simulink model "akgoz_gimbal_stabilized"  (R2025b)
settings: Solver=ode15s  StartTime=0.0  StopTime=12  MaxStep=5e-4  RelTol=1e-5
values from neighbouring files (symbols this model uses):
  kg = gain([a '_kt'],kt(k),[1500 y+120 1550 y+150]); w(is,1,kg,1)    [akgoz_build_controller.m]
  m = akgoz_plot_los(out,['AKGOZ LOS: ' cfg{k,1}])    [akgoz_compare.m]    (also in akgoz_gyro.m = round(m/P.gyro.quant)*P.gyro.quant)
  s = diagSig{r,k}; w(s{1},s{2},dm,n)    [akgoz_build_controller.m]    (also in akgoz_los_kinematics.m = norm(c))
undefined symbols (not defined in the file or in its folder): DiscIntNeverNeededParam, X, Y, Z
libraries: sm_lib x154, nesl_utility x13, simulink x2
(part 1 of 3)
settings Model: Creator=yagiz  LastModifiedBy=yagiz

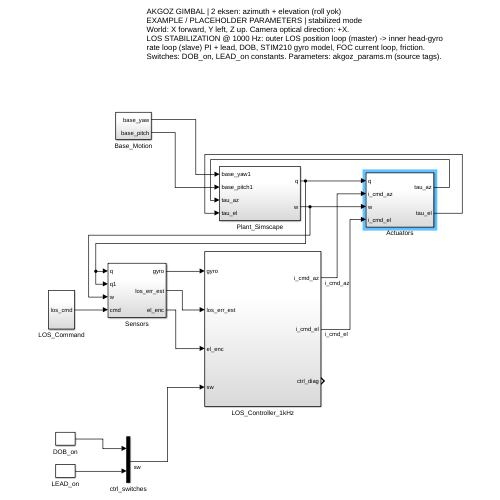
[thumbnail: Simulink's stored preview of the top-level diagram]
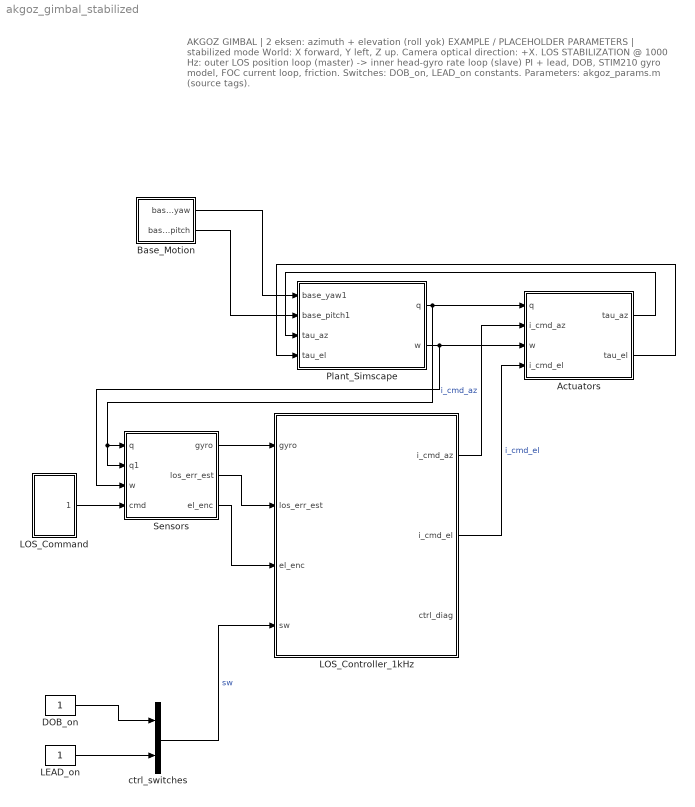
== system akgoz_gimbal_stabilized ==
  note: AKGOZ GIMBAL | 2 eksen: azimuth + elevation (roll yok)
      | EXAMPLE / PLACEHOLDER PARAMETERS | stabilized mode
      | World: X forward, Y left, Z up. Camera optical direction: +X.
      | LOS STABILIZATION @ 1000 Hz: outer LOS position loop (master) -> inner head-gyro
      | rate loop (slave) PI + lead, DOB, STIM210 gyro model, FOC current loop, friction.
      | Switches: DOB_on, LEAD_on constants. Parameters: akgoz_params.m (source tags).
  Actuators : Subsystem
  Base_Motion : Subsystem
  DOB_on : Constant
  LEAD_on : Constant
  LOS_Command : Subsystem
  LOS_Controller_1kHz : Subsystem
  Plant_Simscape : Subsystem
  Sensors : Subsystem
  ctrl_switches : Mux  Inputs=2
  wires:
  DOB_on/1 -> ctrl_switches/1
  LEAD_on/1 -> ctrl_switches/2
  Base_Motion/1(base_yaw) -> Plant_Simscape/1(base_yaw1)
  Actuators/2(tau_el) -> Plant_Simscape/4(tau_el)
  LOS_Command/1(los_cmd) -> Sensors/4(cmd)
  Base_Motion/2(base_pitch) -> Plant_Simscape/2(base_pitch1)
  Sensors/1(gyro) -> LOS_Controller_1kHz/1(gyro)
  Sensors/3(el_enc) -> LOS_Controller_1kHz/3(el_enc)
  Sensors/2(los_err_est) -> LOS_Controller_1kHz/2(los_err_est)
  Plant_Simscape/1(q) -> Sensors/1(q), Sensors/2(q1), Actuators/1(q)
  Plant_Simscape/2(w) -> Actuators/3(w), Sensors/3(w)
  ctrl_switches/1 -> LOS_Controller_1kHz/4(sw)  "sw"
  LOS_Controller_1kHz/1(i_cmd_az) -> Actuators/2(i_cmd_az)  "i_cmd_az"
  Actuators/1(tau_az) -> Plant_Simscape/3(tau_az)
  LOS_Controller_1kHz/2(i_cmd_el) -> Actuators/4(i_cmd_el)  "i_cmd_el"

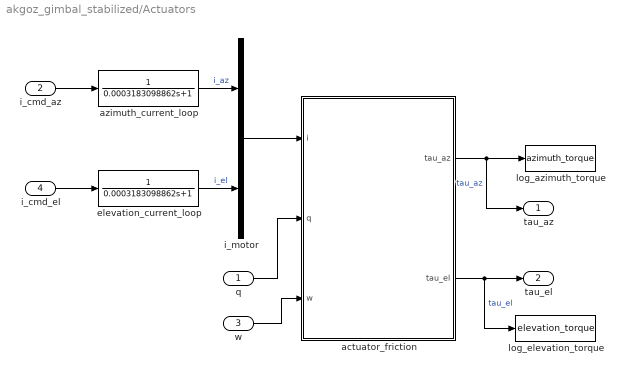
== system akgoz_gimbal_stabilized/Actuators ==
  q : Inport
  i_cmd_az : Inport  Port=2
  w : Inport  Port=3
  i_cmd_el : Inport  Port=4
  actuator_friction : MATLAB Function  TreatAsAtomicUnit=on
  azimuth_current_loop : TransferFcn  Numerator=1  Denominator=[0.0003183098862 1]
  elevation_current_loop : TransferFcn  Numerator=1  Denominator=[0.0003183098862 1]
  i_motor : Mux  Inputs=2
  log_azimuth_torque : ToWorkspace  VariableName=azimuth_torque  SaveFormat=Timeseries  SampleTime=-1
  log_elevation_torque : ToWorkspace  VariableName=elevation_torque  SaveFormat=Timeseries  SampleTime=-1
  tau_az : Outport
  tau_el : Outport  Port=2
  wires:
  actuator_friction/2(tau_el) -> tau_el/1, log_elevation_torque/1  "tau_el"
  actuator_friction/1(tau_az) -> tau_az/1, log_azimuth_torque/1  "tau_az"
  q/1 -> actuator_friction/2(q)
  w/1 -> actuator_friction/3(w)
  i_motor/1 -> actuator_friction/1(i)
  elevation_current_loop/1 -> i_motor/2  "i_el"
  azimuth_current_loop/1 -> i_motor/1  "i_az"
  i_cmd_el/1 -> elevation_current_loop/1
  i_cmd_az/1 -> azimuth_current_loop/1

== system akgoz_gimbal_stabilized/Base_Motion ==
  base_demux : Demux  Outputs=2
  base_motion : MATLAB Function  TreatAsAtomicUnit=on
  clock : Clock
  base_yaw : Outport
  base_pitch : Outport  Port=2
  wires:
  base_demux/2 -> base_pitch/1  "base_pitch"
  base_demux/1 -> base_yaw/1  "base_yaw"
  base_motion/1(y) -> base_demux/1
  clock/1 -> base_motion/1(t)

== system akgoz_gimbal_stabilized/LOS_Command ==
  LOS_az_cmd : Step  Time=6  After=0.2617993877991494  SampleTime=0.001
  LOS_cmd : Mux  Inputs=2
  LOS_el_cmd : Step  Time=2  After=-0.3490658503988659  SampleTime=0.001
  los_cmd : Outport
  wires:
  LOS_cmd/1 -> los_cmd/1  "los_cmd"
  LOS_el_cmd/1 -> LOS_cmd/2
  LOS_az_cmd/1 -> LOS_cmd/1

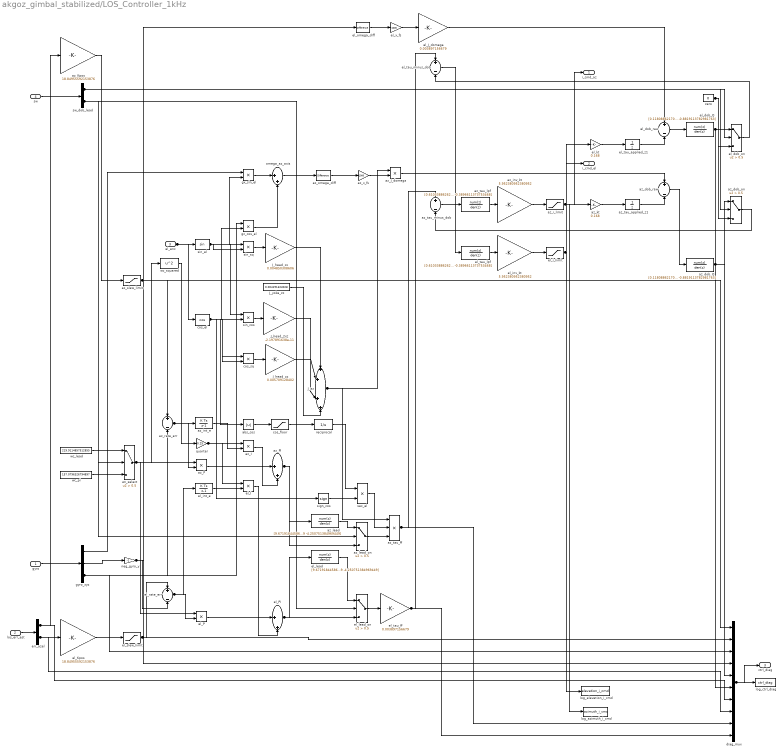
== system akgoz_gimbal_stabilized/LOS_Controller_1kHz ==
  gyro : Inport
  los_err_est : Inport  Port=2
  el_enc : Inport  Port=3
  sw : Inport  Port=4
  J_az : Sum  Inputs=++++
  J_head_2xz : Gain  Gain=-2.197891638e-11
  J_head_xx : Gain  Gain=0.004850308606
  J_head_zz : Gain  Gain=0.005709128402
  J_yoke_zz : Constant  Value=0.004191323028
  abs_cos : Abs  SaturateOnIntegerOverflow=off
  az_I : Product
  az_J_domega : Product
  az_Kpos : Gain  Gain=18.84955592153876
  az_P : Product
  az_PI : Sum  Inputs=|++
  az_dob_Q : DiscreteTransferFcn  Numerator=[0.1180886217018237 0]  Denominator=[1 -0.8819113782981763]  SampleTime=0.001
  az_dob_on : Switch  Criteria=u2 > Threshold  Threshold=0.5  SaturateOnIntegerOverflow=off  InputSameDT=off
  az_dob_raw : Sum  Inputs=+-
  az_i_limit : Saturate  UpperLimit=2.65  LowerLimit=-2.65
  az_int_e : DiscreteIntegrator  SampleTime=0.001  LimitOutput=on  UpperSaturationLimit=0.007289880268834373  LowerSaturationLimit=-0.007289880268834373  ICPrevOutput=DiscIntNeverNeededParam  ICPrevScaledInput=DiscIntNeverNeededParam
  az_inv_kt : Gain  Gain=5.952380952380952
  az_kt : Gain  Gain=0.168
  az_lead : DiscreteTransferFcn  Numerator=[9.671918445869359 -8.517217907490108]  Denominator=[6.250751384969449 -4.250751384969449]  SampleTime=0.001
  az_lead_on : Switch  Criteria=u2 > Threshold  Threshold=0.5  SaturateOnIntegerOverflow=off  InputSameDT=off
  az_omega_diff : simulink/Discrete/Difference  ICPrevInput=0.0  OutMin=[]  OutMax=[]  OutDataType=fixdt(1, 16)  OutScaling=2^-10  DoSatur=off
  az_rate_err : Sum  Inputs=+-
  az_slew_limit : Saturate  UpperLimit=1.047197551196598  LowerLimit=-1.047197551196598
  az_tau_applied_z1 : UnitDelay  SampleTime=0.001  HasFrameUpgradeWarning=on
  az_tau_ff : Product  Inputs=3
  az_tau_lpf : DiscreteTransferFcn  Numerator=[0.6103388626246532 0]  Denominator=[1 -0.3896611373753468]  SampleTime=0.001
  az_tau_minus_dob : Sum  Inputs=+-
  az_x_fs : Gain  Gain=1000
  cos_el : Trigonometry  Operator=cos
  cos_floor : Saturate  UpperLimit=1  LowerLimit=0.2
  cos_sq : Product
  diag_mux : Mux  Inputs=10
  el_I : Product
  el_J_domega : Gain  Gain=0.003897156679
  el_Kpos : Gain  Gain=18.84955592153876
  el_P : Product
  el_PI : Sum  Inputs=|++
  el_dob_Q : DiscreteTransferFcn  Numerator=[0.1180886217018237 0]  Denominator=[1 -0.8819113782981763]  SampleTime=0.001
  el_dob_on : Switch  Criteria=u2 > Threshold  Threshold=0.5  SaturateOnIntegerOverflow=off  InputSameDT=off
  el_dob_raw : Sum  Inputs=+-
  el_i_limit : Saturate  UpperLimit=2.65  LowerLimit=-2.65
  el_int_e : DiscreteIntegrator  SampleTime=0.001  LimitOutput=on  UpperSaturationLimit=0.01851942620655156  LowerSaturationLimit=-0.01851942620655156  ICPrevOutput=DiscIntNeverNeededParam  ICPrevScaledInput=DiscIntNeverNeededParam
  el_inv_kt : Gain  Gain=5.952380952380952
  el_kt : Gain  Gain=0.168
  el_lead : DiscreteTransferFcn  Numerator=[9.671918445869359 -8.517217907490108]  Denominator=[6.250751384969449 -4.250751384969449]  SampleTime=0.001
  el_lead_on : Switch  Criteria=u2 > Threshold  Threshold=0.5  SaturateOnIntegerOverflow=off  InputSameDT=off
  el_omega_diff : simulink/Discrete/Difference  ICPrevInput=0.0  OutMin=[]  OutMax=[]  OutDataType=fixdt(1, 16)  OutScaling=2^-10  DoSatur=off
  el_rate_err : Sum  Inputs=+-
  el_slew_limit : Saturate  UpperLimit=1.047197551196598  LowerLimit=-1.047197551196598
  el_tau_applied_z1 : UnitDelay  SampleTime=0.001  HasFrameUpgradeWarning=on
  el_tau_ff : Gain  Gain=0.003897156679
  el_tau_lpf : DiscreteTransferFcn  Numerator=[0.6103388626246532 0]  Denominator=[1 -0.3896611373753468]  SampleTime=0.001
  el_tau_minus_dob : Sum  Inputs=+-
  el_x_fs : Gain  Gain=1000
  err_azel : Demux  Outputs=2
  gx_sin_el : Product
  gyro_xyz : Demux  Outputs=3
  gz_cos_el : Product
  log_azimuth_i_cmd : ToWorkspace  VariableName=azimuth_i_cmd  SaveFormat=Timeseries  SampleTime=-1
  log_ctrl_diag : ToWorkspace  VariableName=ctrl_diag  SaveFormat=Timeseries  SampleTime=-1
  log_elevation_i_cmd : ToWorkspace  VariableName=elevation_i_cmd  SaveFormat=Timeseries  SampleTime=-1
  neg_gyro_y : Gain  Gain=-1
  omega_az_axis : Sum  Inputs=|++
  quarter : Gain  Gain=0.25
  reciprocal : Math  Operator=reciprocal
  sec_el : Product
  sign_cos : Signum
  sin_cos : Product
  sin_el : Trigonometry
  sin_sq : Product
  sw_dob_lead : Demux  Outputs=2
  wc_lead : Constant  Value=219.9114857512855
  wc_pi : Constant  Value=157.0796326794897
  wc_select : Switch  Criteria=u2 > Threshold  Threshold=0.5  SaturateOnIntegerOverflow=off  InputSameDT=off
  wc_squared : Math  Operator=square
  zero : Constant  Value=0
  i_cmd_az : Outport
  i_cmd_el : Outport  Port=2
  ctrl_diag : Outport  Port=3
  wires:
  diag_mux/1 -> log_ctrl_diag/1, ctrl_diag/1
  az_dob_on/1 -> az_tau_minus_dob/2
  el_dob_on/1 -> el_tau_minus_dob/2
  el_dob_Q/1 -> diag_mux/6, el_dob_on/1
  zero/1 -> el_dob_on/3, az_dob_on/3
  az_dob_raw/1 -> az_dob_Q/1
  el_dob_raw/1 -> el_dob_Q/1
  el_tau_applied_z1/1 -> el_dob_raw/2
  az_kt/1 -> az_tau_applied_z1/1
  el_kt/1 -> el_tau_applied_z1/1
  el_i_limit/1 -> log_elevation_i_cmd/1, el_kt/1, i_cmd_el/1
  el_inv_kt/1 -> el_i_limit/1
  az_inv_kt/1 -> az_i_limit/1
  el_tau_lpf/1 -> el_inv_kt/1
  az_tau_minus_dob/1 -> az_tau_lpf/1
  el_tau_minus_dob/1 -> el_tau_lpf/1
  el_J_domega/1 -> el_dob_raw/1
  el_tau_ff/1 -> el_tau_minus_dob/1, diag_mux/10
  az_P/1 -> az_PI/1
  quarter/1 -> el_I/1, az_I/1
  sin_cos/1 -> J_head_2xz/1
  cos_el/1 -> gz_cos_el/2, abs_cos/1, sin_cos/2, cos_sq/2, cos_sq/1, sign_cos/1
  wc_select/1 -> wc_squared/1, el_P/1, az_P/1
  el_slew_limit/1 -> el_rate_err/1, diag_mux/2
  J_head_zz/1 -> J_az/2
  az_slew_limit/1 -> az_rate_err/1, diag_mux/1
  az_i_limit/1 -> log_azimuth_i_cmd/1, az_kt/1, i_cmd_az/1
  gyro/1 -> gyro_xyz/1
  az_Kpos/1 -> az_slew_limit/1
  az_int_e/1 -> az_I/2
  err_azel/2 -> el_Kpos/1, diag_mux/8
  el_Kpos/1 -> el_slew_limit/1
  los_err_est/1 -> err_azel/1
  el_rate_err/1 -> el_int_e/1, el_P/2
  az_dob_Q/1 -> diag_mux/5, az_dob_on/1
  wc_pi/1 -> wc_select/3
  gyro_xyz/3 -> az_rate_err/2, diag_mux/3, gz_cos_el/1
  wc_squared/1 -> quarter/1
  cos_floor/1 -> reciprocal/1
  az_rate_err/1 -> az_int_e/1, az_P/2
  err_azel/1 -> az_Kpos/1, diag_mux/7
  el_enc/1 -> cos_el/1, sin_el/1
  az_I/1 -> az_PI/2
  el_int_e/1 -> el_I/2
  az_PI/1 -> az_lead/1, az_lead_on/3
  sw_dob_lead/1 -> az_dob_on/2, el_dob_on/2
  sin_el/1 -> gx_sin_el/2, sin_cos/1, sin_sq/2, sin_sq/1
  el_PI/1 -> el_lead/1, el_lead_on/3
  gyro_xyz/2 -> neg_gyro_y/1
  el_omega_diff/1 -> el_x_fs/1
  el_x_fs/1 -> el_J_domega/1
  gx_sin_el/1 -> omega_az_axis/1
  el_lead_on/1 -> el_tau_ff/1
  sw/1 -> sw_dob_lead/1
  az_omega_diff/1 -> az_x_fs/1
  neg_gyro_y/1 -> el_rate_err/2, diag_mux/4, el_omega_diff/1
  sin_sq/1 -> J_head_xx/1
  sw_dob_lead/2 -> wc_select/2, az_lead_on/2, el_lead_on/2
  cos_sq/1 -> J_head_zz/1
  abs_cos/1 -> cos_floor/1
  el_P/1 -> el_PI/1
  el_I/1 -> el_PI/2
  wc_lead/1 -> wc_select/1
  az_tau_ff/1 -> az_tau_minus_dob/1, diag_mux/9
  omega_az_axis/1 -> az_omega_diff/1
  az_tau_lpf/1 -> az_inv_kt/1
  J_head_xx/1 -> J_az/1
  J_yoke_zz/1 -> J_az/4
  J_head_2xz/1 -> J_az/3
  J_az/1 -> az_J_domega/1, az_tau_ff/1
  gyro_xyz/1 -> gx_sin_el/1
  reciprocal/1 -> sec_el/1
  sign_cos/1 -> sec_el/2
  az_lead/1 -> az_lead_on/1
  el_lead/1 -> el_lead_on/1
  gz_cos_el/1 -> omega_az_axis/2
  az_x_fs/1 -> az_J_domega/2
  sec_el/1 -> az_tau_ff/2
  az_lead_on/1 -> az_tau_ff/3
  az_tau_applied_z1/1 -> az_dob_raw/2
  az_J_domega/1 -> az_dob_raw/1

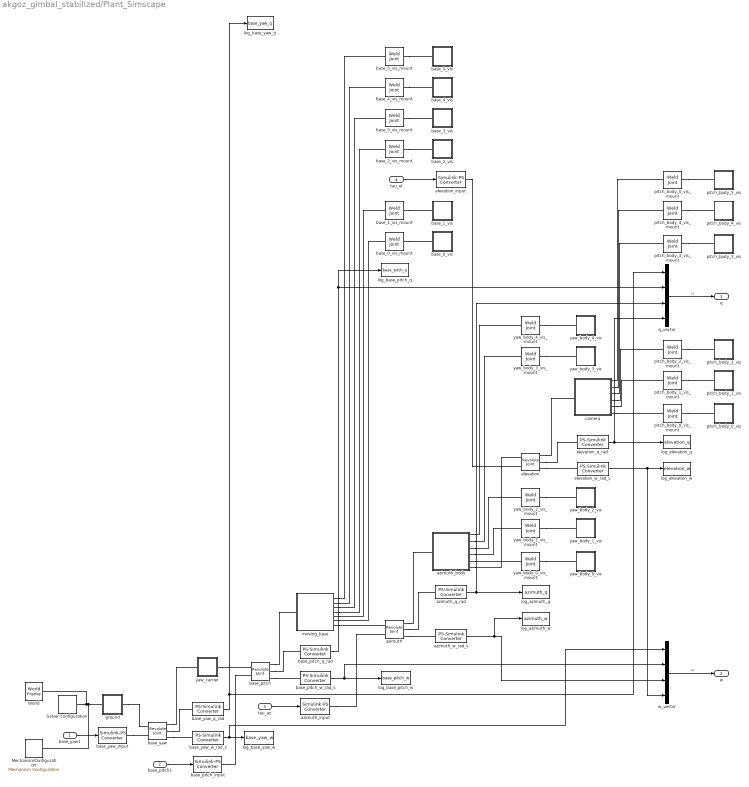
== system akgoz_gimbal_stabilized/Plant_Simscape ==
  base_yaw1 : Inport
  base_pitch1 : Inport  Port=2
  tau_az : Inport  Port=3
  tau_el : Inport  Port=4
  MechanismConfiguration : sm_lib/Utilities/Mechanism Configuration  UniformGravity=Constant  GravityVector=[0 0 -9.80665]  GravityVectorUnits=m/s^2  LinearizationDelta=0.001  JointModeTransitionNonlinearIterations=2
  Solver Configuration : nesl_utility/Solver Configuration  PhysicalDomain=network_engine_domain  SubClassName=solver  LeftPortType=input  RightPortType=generic  Tones=[]  Harmonics=[]  SimulateNoise=off  Profile=off  UseLocalSampling=off  EnableSwitchedLinearOptims=on  FrequencyDomain=off  UseCCode=off  RelTol=0.001  AbsTol=0.001  MinStep=1e-09  ToWorkspace=off  RevertToSquareIcSolve=off  NumHomotopyIterations=100  PhasorMode=off  PhasorModeNumHarmonics=1  ConsistencySolver=NEWTON_XTOL_AFTER_FTOL  IndexReductionMethod=DerivativeReplacement  DoDC=off  ResidualTolerance=1e-09  ConsistencyTolSource=GLOBAL  ConsistencyAbsTol=0.001  ConsistencyRelTol=0.001  ConsistencyTolFactor=0.001  UseLocalSolver=off  LocalSolverChoice=NE_BACKWARD_EULER_ADVANCER  ResolveIndetEquations=on  FunctionEvalNumThread=1  LocalSolverSampleTime=0.001  DoFixedCost=off  MaxNonlinIter=3  MaxModeIter=2  ComputeImpulses=off  ImpulseIterations=2  LinearAlgebra=auto  LinearAlgebraNumThread=0  EquationFormulation=NE_TIME_EF  DelaysMemoryBudget=1024  AutomaticFiltering=on  FilteringTimeConstant=0.001  PartitionStorageMethod=AS_NEEDED  PartitionMemoryBudget=1024  PartitionMethod=ROBUST  MultibodyUseLocalSolver=off  MultibodyLocalSolverChoice=ODE1  MultibodyLocalSolverSampleTime=0.001
  World : sm_lib/Frames and Transforms/World Frame
  azimuth : sm_lib/Joints/Revolute Joint  JointMode=Normal  CompositeWrenchDir=FollowerOnBase  CompositeWrenchFrame=BaseFrame  SenseConstraintForce=off  SenseConstraintTorque=off  SenseTotalForce=off  SenseTotalTorque=off  PositionTargetSpecify=off  PositionTargetPriority=High  PositionTargetValue=0  PositionTargetValueUnits=deg  VelocityTargetSpecify=off  VelocityTargetPriority=High  VelocityTargetValue=0  VelocityTargetValueUnits=deg/s  EquilibriumPosition=0  EquilibriumPositionUnits=deg  SpringStiffness=0  SpringStiffnessUnits=N*m/deg  DampingCoefficient=0  DampingCoefficientUnits=kg*m^2/(rad*s)  LowerLimitSpecify=off  LowerLimitBound=-90  LowerLimitBoundUnits=deg  LowerLimitStiffness=1e4  LowerLimitStiffnessUnits=N*m/deg  LowerLimitDamping=10  LowerLimitDampingUnits=N*m/(deg/s)  LowerLimitTransitionRegionWidth=0.1  LowerLimitTransitionRegionWidthUnits=deg  UpperLimitSpecify=off  UpperLimitBound=90  UpperLimitBoundUnits=deg  UpperLimitStiffness=1e4  UpperLimitStiffnessUnits=N*m/deg  UpperLimitDamping=10  UpperLimitDampingUnits=N*m/(deg/s)  UpperLimitTransitionRegionWidth=0.1  UpperLimitTransitionRegionWidthUnits=deg  TorqueActuationMode=InputTorque  MotionActuationMode=ComputedMotion  SensePosition=on  SenseVelocity=on  SenseAcceleration=off  SenseTorqueForce=off  SenseLowerLimitTorqueForce=off  SenseUpperLimitTorqueForce=off
  azimuth_body : Subsystem
  azimuth_input : nesl_utility/Simulink-PS Converter  PhysicalDomain=network_engine_domain  SubClassName=ps_input  LeftPortType=input  RightPortType=output  PseudoPeriodic=off  Frequencies=[]  NoiseDistribution=none  NoiseParameters=[]  Unit=N*m  AffineConversion=off  FilteringAndDerivatives=provide  SimscapeFilterOrder=1  InputFilterTimeConstant=0.001  UdotUserProvided=0
  azimuth_q_rad : nesl_utility/PS-Simulink Converter  PhysicalDomain=network_engine_domain  SubClassName=ps_output  LeftPortType=input  RightPortType=output  PseudoPeriodic=off  Frequencies=[]  VectorFormat=inherit  Unit=rad  AffineConversion=off
  azimuth_w_rad_s : nesl_utility/PS-Simulink Converter  PhysicalDomain=network_engine_domain  SubClassName=ps_output  LeftPortType=input  RightPortType=output  PseudoPeriodic=off  Frequencies=[]  VectorFormat=inherit  Unit=rad/s  AffineConversion=off
  base_0_vis : Subsystem
  base_0_vis_mount : sm_lib/Joints/Weld Joint  JointMode=Normal  CompositeWrenchDir=FollowerOnBase  CompositeWrenchFrame=BaseFrame  SenseConstraintForce=off  SenseConstraintTorque=off  SenseTotalForce=off  SenseTotalTorque=off
  base_1_vis : Subsystem
  base_1_vis_mount : sm_lib/Joints/Weld Joint  JointMode=Normal  CompositeWrenchDir=FollowerOnBase  CompositeWrenchFrame=BaseFrame  SenseConstraintForce=off  SenseConstraintTorque=off  SenseTotalForce=off  SenseTotalTorque=off
  base_2_vis : Subsystem
  base_2_vis_mount : sm_lib/Joints/Weld Joint  JointMode=Normal  CompositeWrenchDir=FollowerOnBase  CompositeWrenchFrame=BaseFrame  SenseConstraintForce=off  SenseConstraintTorque=off  SenseTotalForce=off  SenseTotalTorque=off
  base_3_vis : Subsystem
  base_3_vis_mount : sm_lib/Joints/Weld Joint  JointMode=Normal  CompositeWrenchDir=FollowerOnBase  CompositeWrenchFrame=BaseFrame  SenseConstraintForce=off  SenseConstraintTorque=off  SenseTotalForce=off  SenseTotalTorque=off
  base_4_vis : Subsystem
  base_4_vis_mount : sm_lib/Joints/Weld Joint  JointMode=Normal  CompositeWrenchDir=FollowerOnBase  CompositeWrenchFrame=BaseFrame  SenseConstraintForce=off  SenseConstraintTorque=off  SenseTotalForce=off  SenseTotalTorque=off
  base_5_vis : Subsystem
  base_5_vis_mount : sm_lib/Joints/Weld Joint  JointMode=Normal  CompositeWrenchDir=FollowerOnBase  CompositeWrenchFrame=BaseFrame  SenseConstraintForce=off  SenseConstraintTorque=off  SenseTotalForce=off  SenseTotalTorque=off
  base_pitch : sm_lib/Joints/Revolute Joint  JointMode=Normal  CompositeWrenchDir=FollowerOnBase  CompositeWrenchFrame=BaseFrame  SenseConstraintForce=off  SenseConstraintTorque=off  SenseTotalForce=off  SenseTotalTorque=off  PositionTargetSpecify=off  PositionTargetPriority=High  PositionTargetValue=0  PositionTargetValueUnits=deg  VelocityTargetSpecify=off  VelocityTargetPriority=High  VelocityTargetValue=0  VelocityTargetValueUnits=deg/s  EquilibriumPosition=0  EquilibriumPositionUnits=deg  SpringStiffness=0  SpringStiffnessUnits=N*m/deg  DampingCoefficient=0  DampingCoefficientUnits=kg*m^2/(rad*s)  LowerLimitSpecify=off  LowerLimitBound=-90  LowerLimitBoundUnits=deg  LowerLimitStiffness=1e4  LowerLimitStiffnessUnits=N*m/deg  LowerLimitDamping=10  LowerLimitDampingUnits=N*m/(deg/s)  LowerLimitTransitionRegionWidth=0.1  LowerLimitTransitionRegionWidthUnits=deg  UpperLimitSpecify=off  UpperLimitBound=90  UpperLimitBoundUnits=deg  UpperLimitStiffness=1e4  UpperLimitStiffnessUnits=N*m/deg  UpperLimitDamping=10  UpperLimitDampingUnits=N*m/(deg/s)  UpperLimitTransitionRegionWidth=0.1  UpperLimitTransitionRegionWidthUnits=deg  TorqueActuationMode=ComputedTorque  MotionActuationMode=InputMotion  SensePosition=on  SenseVelocity=on  SenseAcceleration=off  SenseTorqueForce=off  SenseLowerLimitTorqueForce=off  SenseUpperLimitTorqueForce=off
  base_pitch_input : nesl_utility/Simulink-PS Converter  PhysicalDomain=network_engine_domain  SubClassName=ps_input  LeftPortType=input  RightPortType=output  PseudoPeriodic=off  Frequencies=[]  NoiseDistribution=none  NoiseParameters=[]  Unit=rad  AffineConversion=off  FilteringAndDerivatives=filter  SimscapeFilterOrder=2  InputFilterTimeConstant=5e-4  UdotUserProvided=0
  base_pitch_q_rad : nesl_utility/PS-Simulink Converter  PhysicalDomain=network_engine_domain  SubClassName=ps_output  LeftPortType=input  RightPortType=output  PseudoPeriodic=off  Frequencies=[]  VectorFormat=inherit  Unit=rad  AffineConversion=off
  base_pitch_w_rad_s : nesl_utility/PS-Simulink Converter  PhysicalDomain=network_engine_domain  SubClassName=ps_output  LeftPortType=input  RightPortType=output  PseudoPeriodic=off  Frequencies=[]  VectorFormat=inherit  Unit=rad/s  AffineConversion=off
  base_yaw : sm_lib/Joints/Revolute Joint  JointMode=Normal  CompositeWrenchDir=FollowerOnBase  CompositeWrenchFrame=BaseFrame  SenseConstraintForce=off  SenseConstraintTorque=off  SenseTotalForce=off  SenseTotalTorque=off  PositionTargetSpecify=off  PositionTargetPriority=High  PositionTargetValue=0  PositionTargetValueUnits=deg  VelocityTargetSpecify=off  VelocityTargetPriority=High  VelocityTargetValue=0  VelocityTargetValueUnits=deg/s  EquilibriumPosition=0  EquilibriumPositionUnits=deg  SpringStiffness=0  SpringStiffnessUnits=N*m/deg  DampingCoefficient=0  DampingCoefficientUnits=kg*m^2/(rad*s)  LowerLimitSpecify=off  LowerLimitBound=-90  LowerLimitBoundUnits=deg  LowerLimitStiffness=1e4  LowerLimitStiffnessUnits=N*m/deg  LowerLimitDamping=10  LowerLimitDampingUnits=N*m/(deg/s)  LowerLimitTransitionRegionWidth=0.1  LowerLimitTransitionRegionWidthUnits=deg  UpperLimitSpecify=off  UpperLimitBound=90  UpperLimitBoundUnits=deg  UpperLimitStiffness=1e4  UpperLimitStiffnessUnits=N*m/deg  UpperLimitDamping=10  UpperLimitDampingUnits=N*m/(deg/s)  UpperLimitTransitionRegionWidth=0.1  UpperLimitTransitionRegionWidthUnits=deg  TorqueActuationMode=ComputedTorque  MotionActuationMode=InputMotion  SensePosition=on  SenseVelocity=on  SenseAcceleration=off  SenseTorqueForce=off  SenseLowerLimitTorqueForce=off  SenseUpperLimitTorqueForce=off
  base_yaw_input : nesl_utility/Simulink-PS Converter  PhysicalDomain=network_engine_domain  SubClassName=ps_input  LeftPortType=input  RightPortType=output  PseudoPeriodic=off  Frequencies=[]  NoiseDistribution=none  NoiseParameters=[]  Unit=rad  AffineConversion=off  FilteringAndDerivatives=filter  SimscapeFilterOrder=2  InputFilterTimeConstant=5e-4  UdotUserProvided=0
  base_yaw_q_rad : nesl_utility/PS-Simulink Converter  PhysicalDomain=network_engine_domain  SubClassName=ps_output  LeftPortType=input  RightPortType=output  PseudoPeriodic=off  Frequencies=[]  VectorFormat=inherit  Unit=rad  AffineConversion=off
  base_yaw_w_rad_s : nesl_utility/PS-Simulink Converter  PhysicalDomain=network_engine_domain  SubClassName=ps_output  LeftPortType=input  RightPortType=output  PseudoPeriodic=off  Frequencies=[]  VectorFormat=inherit  Unit=rad/s  AffineConversion=off
  camera : Subsystem
  elevation : sm_lib/Joints/Revolute Joint  JointMode=Normal  CompositeWrenchDir=FollowerOnBase  CompositeWrenchFrame=BaseFrame  SenseConstraintForce=off  SenseConstraintTorque=off  SenseTotalForce=off  SenseTotalTorque=off  PositionTargetSpecify=off  PositionTargetPriority=High  PositionTargetValue=0  PositionTargetValueUnits=deg  VelocityTargetSpecify=off  VelocityTargetPriority=High  VelocityTargetValue=0  VelocityTargetValueUnits=deg/s  EquilibriumPosition=0  EquilibriumPositionUnits=deg  SpringStiffness=0  SpringStiffnessUnits=N*m/deg  DampingCoefficient=0  DampingCoefficientUnits=kg*m^2/(rad*s)  LowerLimitSpecify=off  LowerLimitBound=-90  LowerLimitBoundUnits=deg  LowerLimitStiffness=1e4  LowerLimitStiffnessUnits=N*m/deg  LowerLimitDamping=10  LowerLimitDampingUnits=N*m/(deg/s)  LowerLimitTransitionRegionWidth=0.1  LowerLimitTransitionRegionWidthUnits=deg  UpperLimitSpecify=off  UpperLimitBound=90  UpperLimitBoundUnits=deg  UpperLimitStiffness=1e4  UpperLimitStiffnessUnits=N*m/deg  UpperLimitDamping=10  UpperLimitDampingUnits=N*m/(deg/s)  UpperLimitTransitionRegionWidth=0.1  UpperLimitTransitionRegionWidthUnits=deg  TorqueActuationMode=InputTorque  MotionActuationMode=ComputedMotion  SensePosition=on  SenseVelocity=on  SenseAcceleration=off  SenseTorqueForce=off  SenseLowerLimitTorqueForce=off  SenseUpperLimitTorqueForce=off
  elevation_input : nesl_utility/Simulink-PS Converter  PhysicalDomain=network_engine_domain  SubClassName=ps_input  LeftPortType=input  RightPortType=output  PseudoPeriodic=off  Frequencies=[]  NoiseDistribution=none  NoiseParameters=[]  Unit=N*m  AffineConversion=off  FilteringAndDerivatives=provide  SimscapeFilterOrder=1  InputFilterTimeConstant=0.001  UdotUserProvided=0
  elevation_q_rad : nesl_utility/PS-Simulink Converter  PhysicalDomain=network_engine_domain  SubClassName=ps_output  LeftPortType=input  RightPortType=output  PseudoPeriodic=off  Frequencies=[]  VectorFormat=inherit  Unit=rad  AffineConversion=off
  elevation_w_rad_s : nesl_utility/PS-Simulink Converter  PhysicalDomain=network_engine_domain  SubClassName=ps_output  LeftPortType=input  RightPortType=output  PseudoPeriodic=off  Frequencies=[]  VectorFormat=inherit  Unit=rad/s  AffineConversion=off
  ground : Subsystem
  log_azimuth_q : ToWorkspace  VariableName=azimuth_q  SaveFormat=Timeseries  SampleTime=-1
  log_azimuth_w : ToWorkspace  VariableName=azimuth_w  SaveFormat=Timeseries  SampleTime=-1
  log_base_pitch_q : ToWorkspace  VariableName=base_pitch_q  SaveFormat=Timeseries  SampleTime=-1
  log_base_pitch_w : ToWorkspace  VariableName=base_pitch_w  SaveFormat=Timeseries  SampleTime=-1
  log_base_yaw_q : ToWorkspace  VariableName=base_yaw_q  SaveFormat=Timeseries  SampleTime=-1
  log_base_yaw_w : ToWorkspace  VariableName=base_yaw_w  SaveFormat=Timeseries  SampleTime=-1
  log_elevation_q : ToWorkspace  VariableName=elevation_q  SaveFormat=Timeseries  SampleTime=-1
  log_elevation_w : ToWorkspace  VariableName=elevation_w  SaveFormat=Timeseries  SampleTime=-1
  moving_base : Subsystem
  pitch_body_0_vis : Subsystem
  pitch_body_0_vis_mount : sm_lib/Joints/Weld Joint  JointMode=Normal  CompositeWrenchDir=FollowerOnBase  CompositeWrenchFrame=BaseFrame  SenseConstraintForce=off  SenseConstraintTorque=off  SenseTotalForce=off  SenseTotalTorque=off
  pitch_body_1_vis : Subsystem
  pitch_body_1_vis_mount : sm_lib/Joints/Weld Joint  JointMode=Normal  CompositeWrenchDir=FollowerOnBase  CompositeWrenchFrame=BaseFrame  SenseConstraintForce=off  SenseConstraintTorque=off  SenseTotalForce=off  SenseTotalTorque=off
  pitch_body_2_vis : Subsystem
  pitch_body_2_vis_mount : sm_lib/Joints/Weld Joint  JointMode=Normal  CompositeWrenchDir=FollowerOnBase  CompositeWrenchFrame=BaseFrame  SenseConstraintForce=off  SenseConstraintTorque=off  SenseTotalForce=off  SenseTotalTorque=off
  pitch_body_3_vis : Subsystem
  pitch_body_3_vis_mount : sm_lib/Joints/Weld Joint  JointMode=Normal  CompositeWrenchDir=FollowerOnBase  CompositeWrenchFrame=BaseFrame  SenseConstraintForce=off  SenseConstraintTorque=off  SenseTotalForce=off  SenseTotalTorque=off
  pitch_body_4_vis : Subsystem
  pitch_body_4_vis_mount : sm_lib/Joints/Weld Joint  JointMode=Normal  CompositeWrenchDir=FollowerOnBase  CompositeWrenchFrame=BaseFrame  SenseConstraintForce=off  SenseConstraintTorque=off  SenseTotalForce=off  SenseTotalTorque=off
  pitch_body_5_vis : Subsystem
  pitch_body_5_vis_mount : sm_lib/Joints/Weld Joint  JointMode=Normal  CompositeWrenchDir=FollowerOnBase  CompositeWrenchFrame=BaseFrame  SenseConstraintForce=off  SenseConstraintTorque=off  SenseTotalForce=off  SenseTotalTorque=off
  q_vector : Mux
  w_vector : Mux
  yaw_body_0_vis : Subsystem
  yaw_body_0_vis_mount : sm_lib/Joints/Weld Joint  JointMode=Normal  CompositeWrenchDir=FollowerOnBase  CompositeWrenchFrame=BaseFrame  SenseConstraintForce=off  SenseConstraintTorque=off  SenseTotalForce=off  SenseTotalTorque=off
  yaw_body_1_vis : Subsystem
  yaw_body_1_vis_mount : sm_lib/Joints/Weld Joint  JointMode=Normal  CompositeWrenchDir=FollowerOnBase  CompositeWrenchFrame=BaseFrame  SenseConstraintForce=off  SenseConstraintTorque=off  SenseTotalForce=off  SenseTotalTorque=off
  yaw_body_2_vis : Subsystem
  yaw_body_2_vis_mount : sm_lib/Joints/Weld Joint  JointMode=Normal  CompositeWrenchDir=FollowerOnBase  CompositeWrenchFrame=BaseFrame  SenseConstraintForce=off  SenseConstraintTorque=off  SenseTotalForce=off  SenseTotalTorque=off
  yaw_body_3_vis : Subsystem
  yaw_body_3_vis_mount : sm_lib/Joints/Weld Joint  JointMode=Normal  CompositeWrenchDir=FollowerOnBase  CompositeWrenchFrame=BaseFrame  SenseConstraintForce=off  SenseConstraintTorque=off  SenseTotalForce=off  SenseTotalTorque=off
  yaw_body_4_vis : Subsystem
  yaw_body_4_vis_mount : sm_lib/Joints/Weld Joint  JointMode=Normal  CompositeWrenchDir=FollowerOnBase  CompositeWrenchFrame=BaseFrame  SenseConstraintForce=off  SenseConstraintTorque=off  SenseTotalForce=off  SenseTotalTorque=off
  yaw_carrier : Subsystem
  q : Outport
  w : Outport  Port=2
  wires:
  q_vector/1 -> q/1  "q"
  elevation_w_rad_s/1 -> w_vector/4, log_elevation_w/1
  w_vector/1 -> w/1  "w"
  elevation_q_rad/1 -> q_vector/4, log_elevation_q/1
  base_pitch1/1 -> base_pitch_input/1
  tau_az/1 -> azimuth_input/1
  base_pitch_w_rad_s/1 -> log_base_pitch_w/1, w_vector/2
  base_yaw_q_rad/1 -> log_base_yaw_q/1, q_vector/1
  base_pitch_q_rad/1 -> log_base_pitch_q/1, q_vector/2
  base_yaw_w_rad_s/1 -> log_base_yaw_w/1, w_vector/1
  azimuth_q_rad/1 -> log_azimuth_q/1, q_vector/3
  base_yaw1/1 -> base_yaw_input/1
  tau_el/1 -> elevation_input/1
  azimuth_w_rad_s/1 -> log_azimuth_w/1, w_vector/3
  connections:
  pitch_body_1_vis_mount/RConn1 -- pitch_body_1_vis/LConn1
  pitch_body_3_vis_mount/RConn1 -- pitch_body_3_vis/LConn1
  pitch_body_5_vis_mount/RConn1 -- pitch_body_5_vis/LConn1
  pitch_body_4_vis_mount/RConn1 -- pitch_body_4_vis/LConn1
  moving_base/RConn1 -- base_5_vis_mount/LConn1
  moving_base/RConn2 -- base_4_vis_mount/LConn1
  base_3_vis_mount/RConn1 -- base_3_vis/LConn1
  base_pitch_input/RConn1 -- base_pitch/LConn2
  moving_base/RConn6 -- base_0_vis_mount/LConn1
  moving_base/RConn4 -- base_2_vis_mount/LConn1
  azimuth_body/RConn3 -- yaw_body_2_vis_mount/LConn1
  moving_base/RConn7 -- azimuth/LConn1
  base_pitch/RConn3 -- base_pitch_w_rad_s/LConn1
  elevation_input/RConn1 -- elevation/LConn2
  Solver Configuration/RConn1 -- ground/LConn1 -- MechanismConfiguration/RConn1 -- World/RConn1
  base_4_vis_mount/RConn1 -- base_4_vis/LConn1
  moving_base/RConn5 -- base_1_vis_mount/LConn1
  base_1_vis_mount/RConn1 -- base_1_vis/LConn1
  yaw_carrier/RConn1 -- base_pitch/LConn1
  camera/RConn2 -- pitch_body_4_vis_mount/LConn1
  base_5_vis_mount/RConn1 -- base_5_vis/LConn1
  base_0_vis_mount/RConn1 -- base_0_vis/LConn1
  base_yaw_input/RConn1 -- base_yaw/LConn2
  base_pitch/RConn1 -- moving_base/LConn1
  azimuth_body/RConn5 -- yaw_body_0_vis_mount/LConn1
  base_yaw/RConn3 -- base_yaw_w_rad_s/LConn1
  camera/RConn3 -- pitch_body_3_vis_mount/LConn1
  moving_base/RConn3 -- base_3_vis_mount/LConn1
  azimuth_input/RConn1 -- azimuth/LConn2
  ground/RConn1 -- base_yaw/LConn1
  base_yaw/RConn1 -- yaw_carrier/LConn1
  pitch_body_2_vis_mount/RConn1 -- pitch_body_2_vis/LConn1
  elevation/RConn2 -- elevation_q_rad/LConn1
  camera/RConn1 -- pitch_body_5_vis_mount/LConn1
  base_yaw/RConn2 -- base_yaw_q_rad/LConn1
  base_pitch/RConn2 -- base_pitch_q_rad/LConn1
  azimuth/RConn2 -- azimuth_q_rad/LConn1
  yaw_body_4_vis_mount/RConn1 -- yaw_body_4_vis/LConn1
  azimuth_body/RConn1 -- yaw_body_4_vis_mount/LConn1
  pitch_body_0_vis_mount/RConn1 -- pitch_body_0_vis/LConn1
  yaw_body_2_vis_mount/RConn1 -- yaw_body_2_vis/LConn1
  elevation/RConn3 -- elevation_w_rad_s/LConn1
  azimuth/RConn3 -- azimuth_w_rad_s/LConn1
  azimuth_body/RConn2 -- yaw_body_3_vis_mount/LConn1
  camera/RConn5 -- pitch_body_1_vis_mount/LConn1
  azimuth_body/RConn4 -- yaw_body_1_vis_mount/LConn1
  azimuth_body/RConn6 -- elevation/LConn1
  yaw_body_3_vis_mount/RConn1 -- yaw_body_3_vis/LConn1
  camera/RConn4 -- pitch_body_2_vis_mount/LConn1
  base_2_vis_mount/RConn1 -- base_2_vis/LConn1
  camera/RConn6 -- pitch_body_0_vis_mount/LConn1
  elevation/RConn1 -- camera/LConn1
  yaw_body_1_vis_mount/RConn1 -- yaw_body_1_vis/LConn1
  azimuth/RConn1 -- azimuth_body/LConn1
  yaw_body_0_vis_mount/RConn1 -- yaw_body_0_vis/LConn1

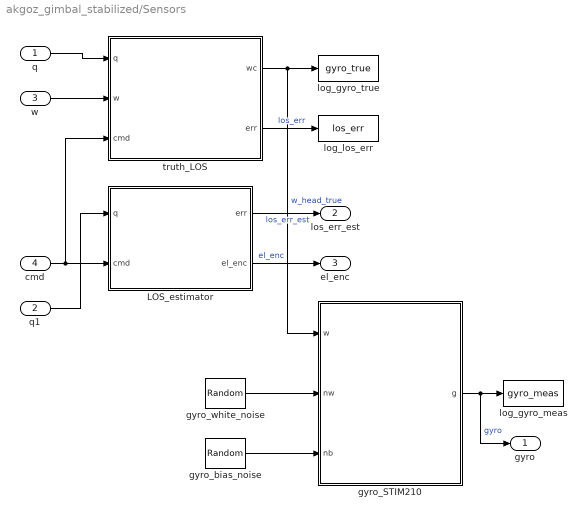
== system akgoz_gimbal_stabilized/Sensors ==
  q : Inport
  q1 : Inport  Port=2
  w : Inport  Port=3
  cmd : Inport  Port=4
  LOS_estimator : MATLAB Function  TreatAsAtomicUnit=on
  gyro_STIM210 : MATLAB Function  TreatAsAtomicUnit=on
  gyro_bias_noise : RandomNumber  Mean=[0 0 0]  Variance=[1 1 1]  Seed=[21 22 23]  SampleTime=0.001
  gyro_white_noise : RandomNumber  Mean=[0 0 0]  Variance=[1 1 1]  Seed=[11 12 13]  SampleTime=0.001
  log_gyro_meas : ToWorkspace  VariableName=gyro_meas  SaveFormat=Timeseries  SampleTime=-1
  log_gyro_true : ToWorkspace  VariableName=gyro_true  SaveFormat=Timeseries  SampleTime=-1
  log_los_err : ToWorkspace  VariableName=los_err  SaveFormat=Timeseries  SampleTime=-1
  truth_LOS : MATLAB Function  TreatAsAtomicUnit=on
  gyro : Outport
  los_err_est : Outport  Port=2
  el_enc : Outport  Port=3
  wires:
  gyro_STIM210/1(g) -> gyro/1, log_gyro_meas/1  "gyro"
  gyro_white_noise/1 -> gyro_STIM210/2(nw)
  truth_LOS/1(wc) -> gyro_STIM210/1(w), log_gyro_true/1  "w_head_true"
  gyro_bias_noise/1 -> gyro_STIM210/3(nb)
  LOS_estimator/2(el_enc) -> el_enc/1  "el_enc"
  LOS_estimator/1(err) -> los_err_est/1  "los_err_est"
  q1/1 -> LOS_estimator/1(q)
  cmd/1 -> LOS_estimator/2(cmd), truth_LOS/3(cmd)
  w/1 -> truth_LOS/2(w)
  truth_LOS/2(err) -> log_los_err/1  "los_err"
  q/1 -> truth_LOS/1(q)

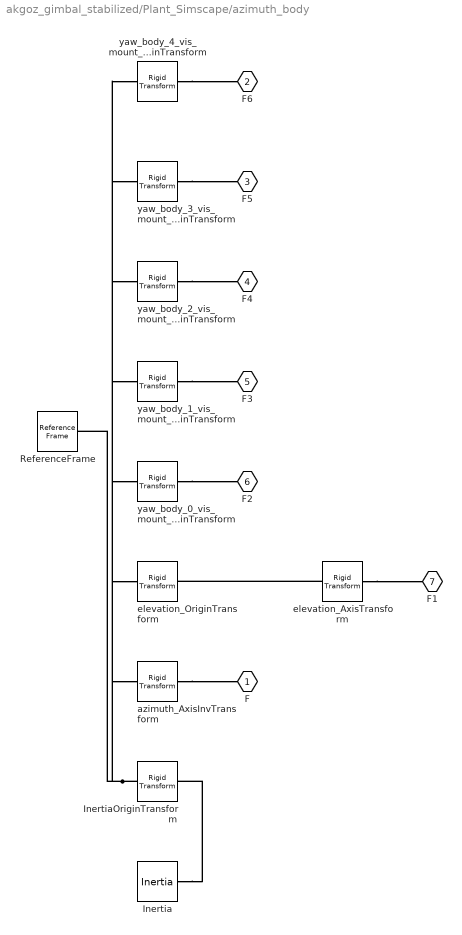
== system akgoz_gimbal_stabilized/Plant_Simscape/azimuth_body ==
  Inertia : sm_lib/Body Elements/Inertia  InertiaType=Custom  Mass=0.6424421311  MassUnits=kg  CenterOfMass=[0, 0, 0]  CenterOfMassUnits=m  MomentsOfInertia=[0.005843944708, 0.00205898437, 0.004161459031]  MomentsOfInertiaUnits=kg*m^2  ProductsOfInertia=[-0.0004493716263, 1.420739885e-21, -1.70053407e-19]  ProductsOfInertiaUnits=kg*m^2  GraphicType=None  MarkerShape=Inertia  MarkerSize=20  GraphicVisPropType=SimpleVisualProperties  GraphicDiffuseColor=[0.5 0.5 0.5]  GraphicOpacity=1  GraphicSpecularColor=[0.5 0.5 0.5 1.0]  GraphicAmbientColor=[0.15 0.15 0.15 1.0]  GraphicEmissiveColor=[0.0 0.0 0.0 1.0]  GraphicShininess=75
  InertiaOriginTransform : sm_lib/Frames and Transforms/Rigid Transform  RotationMethod=RotationSequence  FollAlignAxisA=+X  BaseAlignAxisA=+Y  FollAlignAxisB=+Y  BaseAlignAxisB=+Z  RotationStandardAxis=+Z  RotationAngle=0  RotationAngleUnits=deg  RotationArbitraryAxis=[0 0 1]  RotationSequenceAxes=BaseAxes  RotationSequence=XYZ  RotationSequenceAngles=[0, 0, 0]  RotationSequenceAnglesUnits=rad  RotationMatrix=[1 0 0;0 1 0;0 0 1]  Quaternion=[1 0 0 0]  TranslationMethod=Cartesian  TranslationCartesianOffset=[9.212909614e-19, -0.006817999421, 0.04823722791]  TranslationCartesianOffsetUnits=m  TranslationStandardAxis=+Z  TranslationStandardOffset=0  TranslationStandardOffsetUnits=m  TranslationROffset=0  TranslationROffsetUnits=m  TranslationThetaOffset=0  TranslationThetaOffsetUnits=deg  TranslationZOffset=0  TranslationZOffsetUnits=m
  ReferenceFrame : sm_lib/Frames and Transforms/Reference Frame
  azimuth_AxisInvTransform : sm_lib/Frames and Transforms/Rigid Transform  RotationMethod=ArbitraryAxis  FollAlignAxisA=+X  BaseAlignAxisA=+Y  FollAlignAxisB=+Y  BaseAlignAxisB=+Z  RotationStandardAxis=+Z  RotationAngle=0  RotationAngleUnits=rad  RotationArbitraryAxis=[1, 0, 0]  RotationSequenceAxes=FollowerAxes  RotationSequence=XYX  RotationSequenceAngles=[0 0 0]  RotationSequenceAnglesUnits=deg  RotationMatrix=[1 0 0;0 1 0;0 0 1]  Quaternion=[1 0 0 0]  TranslationMethod=Cartesian  TranslationCartesianOffset=[0, 0, 0]  TranslationCartesianOffsetUnits=m  TranslationStandardAxis=+Z  TranslationStandardOffset=0  TranslationStandardOffsetUnits=m  TranslationROffset=0  TranslationROffsetUnits=m  TranslationThetaOffset=0  TranslationThetaOffsetUnits=deg  TranslationZOffset=0  TranslationZOffsetUnits=m
  elevation_AxisTransform : sm_lib/Frames and Transforms/Rigid Transform  RotationMethod=ArbitraryAxis  FollAlignAxisA=+X  BaseAlignAxisA=+Y  FollAlignAxisB=+Y  BaseAlignAxisB=+Z  RotationStandardAxis=+Z  RotationAngle=1.570796326794897  RotationAngleUnits=rad  RotationArbitraryAxis=[1, 0, 0]  RotationSequenceAxes=FollowerAxes  RotationSequence=XYX  RotationSequenceAngles=[0 0 0]  RotationSequenceAnglesUnits=deg  RotationMatrix=[1 0 0;0 1 0;0 0 1]  Quaternion=[1 0 0 0]  TranslationMethod=Cartesian  TranslationCartesianOffset=[0, 0, 0]  TranslationCartesianOffsetUnits=m  TranslationStandardAxis=+Z  TranslationStandardOffset=0  TranslationStandardOffsetUnits=m  TranslationROffset=0  TranslationROffsetUnits=m  TranslationThetaOffset=0  TranslationThetaOffsetUnits=deg  TranslationZOffset=0  TranslationZOffsetUnits=m
  elevation_OriginTransform : sm_lib/Frames and Transforms/Rigid Transform  RotationMethod=RotationSequence  FollAlignAxisA=+X  BaseAlignAxisA=+Y  FollAlignAxisB=+Y  BaseAlignAxisB=+Z  RotationStandardAxis=+Z  RotationAngle=0  RotationAngleUnits=deg  RotationArbitraryAxis=[0 0 1]  RotationSequenceAxes=BaseAxes  RotationSequence=XYZ  RotationSequenceAngles=[0, 0, 0]  RotationSequenceAnglesUnits=rad  RotationMatrix=[1 0 0;0 1 0;0 0 1]  Quaternion=[1 0 0 0]  TranslationMethod=Cartesian  TranslationCartesianOffset=[0, 0, 0]  TranslationCartesianOffsetUnits=m  TranslationStandardAxis=+Z  TranslationStandardOffset=0  TranslationStandardOffsetUnits=m  TranslationROffset=0  TranslationROffsetUnits=m  TranslationThetaOffset=0  TranslationThetaOffsetUnits=deg  TranslationZOffset=0  TranslationZOffsetUnits=m
  yaw_body_0_vis_mount_OriginTransform : sm_lib/Frames and Transforms/Rigid Transform  RotationMethod=RotationSequence  FollAlignAxisA=+X  BaseAlignAxisA=+Y  FollAlignAxisB=+Y  BaseAlignAxisB=+Z  RotationStandardAxis=+Z  RotationAngle=0  RotationAngleUnits=deg  RotationArbitraryAxis=[0 0 1]  RotationSequenceAxes=BaseAxes  RotationSequence=XYZ  RotationSequenceAngles=[0, 0, 0]  RotationSequenceAnglesUnits=rad  RotationMatrix=[1 0 0;0 1 0;0 0 1]  Quaternion=[1 0 0 0]  TranslationMethod=Cartesian  TranslationCartesianOffset=[0, 0, 0]  TranslationCartesianOffsetUnits=m  TranslationStandardAxis=+Z  TranslationStandardOffset=0  TranslationStandardOffsetUnits=m  TranslationROffset=0  TranslationROffsetUnits=m  TranslationThetaOffset=0  TranslationThetaOffsetUnits=deg  TranslationZOffset=0  TranslationZOffsetUnits=m
  yaw_body_1_vis_mount_OriginTransform : sm_lib/Frames and Transforms/Rigid Transform  RotationMethod=RotationSequence  FollAlignAxisA=+X  BaseAlignAxisA=+Y  FollAlignAxisB=+Y  BaseAlignAxisB=+Z  RotationStandardAxis=+Z  RotationAngle=0  RotationAngleUnits=deg  RotationArbitraryAxis=[0 0 1]  RotationSequenceAxes=BaseAxes  RotationSequence=XYZ  RotationSequenceAngles=[0, 0, 0]  RotationSequenceAnglesUnits=rad  RotationMatrix=[1 0 0;0 1 0;0 0 1]  Quaternion=[1 0 0 0]  TranslationMethod=Cartesian  TranslationCartesianOffset=[0, 0, 0]  TranslationCartesianOffsetUnits=m  TranslationStandardAxis=+Z  TranslationStandardOffset=0  TranslationStandardOffsetUnits=m  TranslationROffset=0  TranslationROffsetUnits=m  TranslationThetaOffset=0  TranslationThetaOffsetUnits=deg  TranslationZOffset=0  TranslationZOffsetUnits=m
  yaw_body_2_vis_mount_OriginTransform : sm_lib/Frames and Transforms/Rigid Transform  RotationMethod=RotationSequence  FollAlignAxisA=+X  BaseAlignAxisA=+Y  FollAlignAxisB=+Y  BaseAlignAxisB=+Z  RotationStandardAxis=+Z  RotationAngle=0  RotationAngleUnits=deg  RotationArbitraryAxis=[0 0 1]  RotationSequenceAxes=BaseAxes  RotationSequence=XYZ  RotationSequenceAngles=[0, 0, 0]  RotationSequenceAnglesUnits=rad  RotationMatrix=[1 0 0;0 1 0;0 0 1]  Quaternion=[1 0 0 0]  TranslationMethod=Cartesian  TranslationCartesianOffset=[0, 0, 0]  TranslationCartesianOffsetUnits=m  TranslationStandardAxis=+Z  TranslationStandardOffset=0  TranslationStandardOffsetUnits=m  TranslationROffset=0  TranslationROffsetUnits=m  TranslationThetaOffset=0  TranslationThetaOffsetUnits=deg  TranslationZOffset=0  TranslationZOffsetUnits=m
  yaw_body_3_vis_mount_OriginTransform : sm_lib/Frames and Transforms/Rigid Transform  RotationMethod=RotationSequence  FollAlignAxisA=+X  BaseAlignAxisA=+Y  FollAlignAxisB=+Y  BaseAlignAxisB=+Z  RotationStandardAxis=+Z  RotationAngle=0  RotationAngleUnits=deg  RotationArbitraryAxis=[0 0 1]  RotationSequenceAxes=BaseAxes  RotationSequence=XYZ  RotationSequenceAngles=[0, 0, 0]  RotationSequenceAnglesUnits=rad  RotationMatrix=[1 0 0;0 1 0;0 0 1]  Quaternion=[1 0 0 0]  TranslationMethod=Cartesian  TranslationCartesianOffset=[0, 0, 0]  TranslationCartesianOffsetUnits=m  TranslationStandardAxis=+Z  TranslationStandardOffset=0  TranslationStandardOffsetUnits=m  TranslationROffset=0  TranslationROffsetUnits=m  TranslationThetaOffset=0  TranslationThetaOffsetUnits=deg  TranslationZOffset=0  TranslationZOffsetUnits=m
  yaw_body_4_vis_mount_OriginTransform : sm_lib/Frames and Transforms/Rigid Transform  RotationMethod=RotationSequence  FollAlignAxisA=+X  BaseAlignAxisA=+Y  FollAlignAxisB=+Y  BaseAlignAxisB=+Z  RotationStandardAxis=+Z  RotationAngle=0  RotationAngleUnits=deg  RotationArbitraryAxis=[0 0 1]  RotationSequenceAxes=BaseAxes  RotationSequence=XYZ  RotationSequenceAngles=[0, 0, 0]  RotationSequenceAnglesUnits=rad  RotationMatrix=[1 0 0;0 1 0;0 0 1]  Quaternion=[1 0 0 0]  TranslationMethod=Cartesian  TranslationCartesianOffset=[0, 0, 0]  TranslationCartesianOffsetUnits=m  TranslationStandardAxis=+Z  TranslationStandardOffset=0  TranslationStandardOffsetUnits=m  TranslationROffset=0  TranslationROffsetUnits=m  TranslationThetaOffset=0  TranslationThetaOffsetUnits=deg  TranslationZOffset=0  TranslationZOffsetUnits=m
  F : PMIOPort  Side=Left
  F6 : PMIOPort  Port=2  Side=Right
  F5 : PMIOPort  Port=3  Side=Right
  F4 : PMIOPort  Port=4  Side=Right
  F3 : PMIOPort  Port=5  Side=Right
  F2 : PMIOPort  Port=6  Side=Right
  F1 : PMIOPort  Port=7  Side=Right
  connections:
  Inertia/RConn1 -- InertiaOriginTransform/RConn1
  ReferenceFrame/RConn1 -- InertiaOriginTransform/LConn1 -- azimuth_AxisInvTransform/LConn1 -- elevation_OriginTransform/LConn1 -- yaw_body_0_vis_mount_OriginTransform/LConn1 -- yaw_body_1_vis_mount_OriginTransform/LConn1 -- yaw_body_2_vis_mount_OriginTransform/LConn1 -- yaw_body_3_vis_mount_OriginTransform/LConn1 -- yaw_body_4_vis_mount_OriginTransform/LConn1
  azimuth_AxisInvTransform/RConn1 -- F/RConn1
  elevation_AxisTransform/RConn1 -- F1/RConn1
  elevation_AxisTransform/LConn1 -- elevation_OriginTransform/RConn1
  yaw_body_0_vis_mount_OriginTransform/RConn1 -- F2/RConn1
  yaw_body_1_vis_mount_OriginTransform/RConn1 -- F3/RConn1
  yaw_body_2_vis_mount_OriginTransform/RConn1 -- F4/RConn1
  yaw_body_3_vis_mount_OriginTransform/RConn1 -- F5/RConn1
  yaw_body_4_vis_mount_OriginTransform/RConn1 -- F6/RConn1

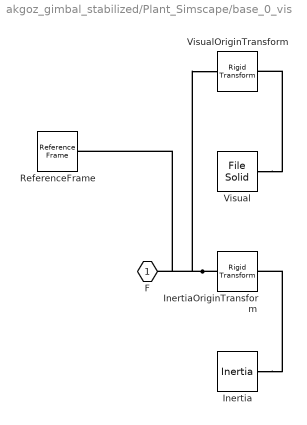
== system akgoz_gimbal_stabilized/Plant_Simscape/base_0_vis ==
  Inertia : sm_lib/Body Elements/Inertia  InertiaType=Custom  Mass=1e-06  MassUnits=kg  CenterOfMass=[0, 0, 0]  CenterOfMassUnits=m  MomentsOfInertia=[1e-12, 1e-12, 1e-12]  MomentsOfInertiaUnits=kg*m^2  ProductsOfInertia=[0, 0, 0]  ProductsOfInertiaUnits=kg*m^2  GraphicType=None  MarkerShape=Inertia  MarkerSize=20  GraphicVisPropType=SimpleVisualProperties  GraphicDiffuseColor=[0.5 0.5 0.5]  GraphicOpacity=1  GraphicSpecularColor=[0.5 0.5 0.5 1.0]  GraphicAmbientColor=[0.15 0.15 0.15 1.0]  GraphicEmissiveColor=[0.0 0.0 0.0 1.0]  GraphicShininess=75
  InertiaOriginTransform : sm_lib/Frames and Transforms/Rigid Transform  RotationMethod=RotationSequence  FollAlignAxisA=+X  BaseAlignAxisA=+Y  FollAlignAxisB=+Y  BaseAlignAxisB=+Z  RotationStandardAxis=+Z  RotationAngle=0  RotationAngleUnits=deg  RotationArbitraryAxis=[0 0 1]  RotationSequenceAxes=BaseAxes  RotationSequence=XYZ  RotationSequenceAngles=[0, 0, 0]  RotationSequenceAnglesUnits=rad  RotationMatrix=[1 0 0;0 1 0;0 0 1]  Quaternion=[1 0 0 0]  TranslationMethod=Cartesian  TranslationCartesianOffset=[0, 0, 0]  TranslationCartesianOffsetUnits=m  TranslationStandardAxis=+Z  TranslationStandardOffset=0  TranslationStandardOffsetUnits=m  TranslationROffset=0  TranslationROffsetUnits=m  TranslationThetaOffset=0  TranslationThetaOffsetUnits=deg  TranslationZOffset=0  TranslationZOffsetUnits=m
  ReferenceFrame : sm_lib/Frames and Transforms/Reference Frame
  Visual : sm_lib/Body Elements/File Solid  ExtGeomFileName=meshes/cad/base_0.stl  UnitType=Custom  ExtGeomFileUnits=m  StepReaderType=HEX  ExportConvexHullGeometry=off  InertiaType=Custom  BasedOnType=DensityFromFile  Density=1000  DensityUnits=kg/m^3  Mass=0  MassUnits=kg  CenterOfMass=[0, 0, 0]  CenterOfMassUnits=m  MomentsOfInertia=[0, 0, 0]  MomentsOfInertiaUnits=kg*m^2  ProductsOfInertia=[0, 0, 0]  ProductsOfInertiaUnits=kg*m^2  GraphicType=FromGeometry  MarkerShape=Sphere  MarkerSize=10  GraphicVisPropType=SimpleVisualProperties  GraphicDiffuseColor=[0.05, 0.05, 0.05]  GraphicOpacity=1  GraphicSpecularColor=[0.5 0.5 0.5 1.0]  GraphicAmbientColor=[0.15 0.15 0.15 1.0]  GraphicEmissiveColor=[0.0 0.0 0.0 1.0]  GraphicShininess=75  DoExposeReferenceFrame=on  SerializedFrames=<Frames/>
  VisualOriginTransform : sm_lib/Frames and Transforms/Rigid Transform  RotationMethod=RotationSequence  FollAlignAxisA=+X  BaseAlignAxisA=+Y  FollAlignAxisB=+Y  BaseAlignAxisB=+Z  RotationStandardAxis=+Z  RotationAngle=0  RotationAngleUnits=deg  RotationArbitraryAxis=[0 0 1]  RotationSequenceAxes=BaseAxes  RotationSequence=XYZ  RotationSequenceAngles=[0, 0, 0]  RotationSequenceAnglesUnits=rad  RotationMatrix=[1 0 0;0 1 0;0 0 1]  Quaternion=[1 0 0 0]  TranslationMethod=Cartesian  TranslationCartesianOffset=[0, 0, -0.186047]  TranslationCartesianOffsetUnits=m  TranslationStandardAxis=+Z  TranslationStandardOffset=0  TranslationStandardOffsetUnits=m  TranslationROffset=0  TranslationROffsetUnits=m  TranslationThetaOffset=0  TranslationThetaOffsetUnits=deg  TranslationZOffset=0  TranslationZOffsetUnits=m
  F : PMIOPort  Side=Left
  connections:
  Inertia/RConn1 -- InertiaOriginTransform/RConn1
  ReferenceFrame/RConn1 -- InertiaOriginTransform/LConn1 -- VisualOriginTransform/LConn1 -- F/RConn1
  Visual/RConn1 -- VisualOriginTransform/RConn1

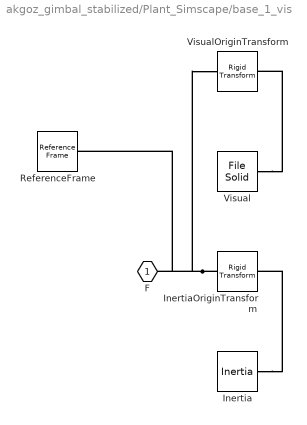
== system akgoz_gimbal_stabilized/Plant_Simscape/base_1_vis ==
  Inertia : sm_lib/Body Elements/Inertia  InertiaType=Custom  Mass=1e-06  MassUnits=kg  CenterOfMass=[0, 0, 0]  CenterOfMassUnits=m  MomentsOfInertia=[1e-12, 1e-12, 1e-12]  MomentsOfInertiaUnits=kg*m^2  ProductsOfInertia=[0, 0, 0]  ProductsOfInertiaUnits=kg*m^2  GraphicType=None  MarkerShape=Inertia  MarkerSize=20  GraphicVisPropType=SimpleVisualProperties  GraphicDiffuseColor=[0.5 0.5 0.5]  GraphicOpacity=1  GraphicSpecularColor=[0.5 0.5 0.5 1.0]  GraphicAmbientColor=[0.15 0.15 0.15 1.0]  GraphicEmissiveColor=[0.0 0.0 0.0 1.0]  GraphicShininess=75
  InertiaOriginTransform : sm_lib/Frames and Transforms/Rigid Transform  RotationMethod=RotationSequence  FollAlignAxisA=+X  BaseAlignAxisA=+Y  FollAlignAxisB=+Y  BaseAlignAxisB=+Z  RotationStandardAxis=+Z  RotationAngle=0  RotationAngleUnits=deg  RotationArbitraryAxis=[0 0 1]  RotationSequenceAxes=BaseAxes  RotationSequence=XYZ  RotationSequenceAngles=[0, 0, 0]  RotationSequenceAnglesUnits=rad  RotationMatrix=[1 0 0;0 1 0;0 0 1]  Quaternion=[1 0 0 0]  TranslationMethod=Cartesian  TranslationCartesianOffset=[0, 0, 0]  TranslationCartesianOffsetUnits=m  TranslationStandardAxis=+Z  TranslationStandardOffset=0  TranslationStandardOffsetUnits=m  TranslationROffset=0  TranslationROffsetUnits=m  TranslationThetaOffset=0  TranslationThetaOffsetUnits=deg  TranslationZOffset=0  TranslationZOffsetUnits=m
  ReferenceFrame : sm_lib/Frames and Transforms/Reference Frame
  Visual : sm_lib/Body Elements/File Solid  ExtGeomFileName=meshes/cad/base_1.stl  UnitType=Custom  ExtGeomFileUnits=m  StepReaderType=HEX  ExportConvexHullGeometry=off  InertiaType=Custom  BasedOnType=DensityFromFile  Density=1000  DensityUnits=kg/m^3  Mass=0  MassUnits=kg  CenterOfMass=[0, 0, 0]  CenterOfMassUnits=m  MomentsOfInertia=[0, 0, 0]  MomentsOfInertiaUnits=kg*m^2  ProductsOfInertia=[0, 0, 0]  ProductsOfInertiaUnits=kg*m^2  GraphicType=FromGeometry  MarkerShape=Sphere  MarkerSize=10  GraphicVisPropType=SimpleVisualProperties  GraphicDiffuseColor=[0.1, 0.45, 0.15]  GraphicOpacity=1  GraphicSpecularColor=[0.5 0.5 0.5 1.0]  GraphicAmbientColor=[0.15 0.15 0.15 1.0]  GraphicEmissiveColor=[0.0 0.0 0.0 1.0]  GraphicShininess=75  DoExposeReferenceFrame=on  SerializedFrames=<Frames/>
  VisualOriginTransform : sm_lib/Frames and Transforms/Rigid Transform  RotationMethod=RotationSequence  FollAlignAxisA=+X  BaseAlignAxisA=+Y  FollAlignAxisB=+Y  BaseAlignAxisB=+Z  RotationStandardAxis=+Z  RotationAngle=0  RotationAngleUnits=deg  RotationArbitraryAxis=[0 0 1]  RotationSequenceAxes=BaseAxes  RotationSequence=XYZ  RotationSequenceAngles=[0, 0, 0]  RotationSequenceAnglesUnits=rad  RotationMatrix=[1 0 0;0 1 0;0 0 1]  Quaternion=[1 0 0 0]  TranslationMethod=Cartesian  TranslationCartesianOffset=[0, 0, -0.186047]  TranslationCartesianOffsetUnits=m  TranslationStandardAxis=+Z  TranslationStandardOffset=0  TranslationStandardOffsetUnits=m  TranslationROffset=0  TranslationROffsetUnits=m  TranslationThetaOffset=0  TranslationThetaOffsetUnits=deg  TranslationZOffset=0  TranslationZOffsetUnits=m
  F : PMIOPort  Side=Left
  connections:
  Inertia/RConn1 -- InertiaOriginTransform/RConn1
  ReferenceFrame/RConn1 -- InertiaOriginTransform/LConn1 -- VisualOriginTransform/LConn1 -- F/RConn1
  Visual/RConn1 -- VisualOriginTransform/RConn1
